simulink model "HVAC_ROS2_SafeSetpoint_v1"  (R2022b)
settings: Solver=FixedStepDiscrete  StartTime=0  StopTime=75  FixedStep=0.1  RelTol=1e-3
libraries: ros2lib x17
settings Model: Creator=Utilisateur  LastModifiedBy=Utilisateur
settings DataIOCC: ReturnWorkspaceOutputs=off
settings OptimizationCC: UseDivisionForNetSlopeComputation=on

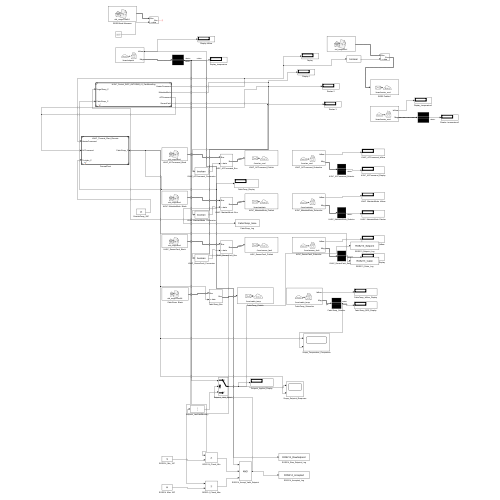
[thumbnail: Simulink's stored preview of the top-level diagram]
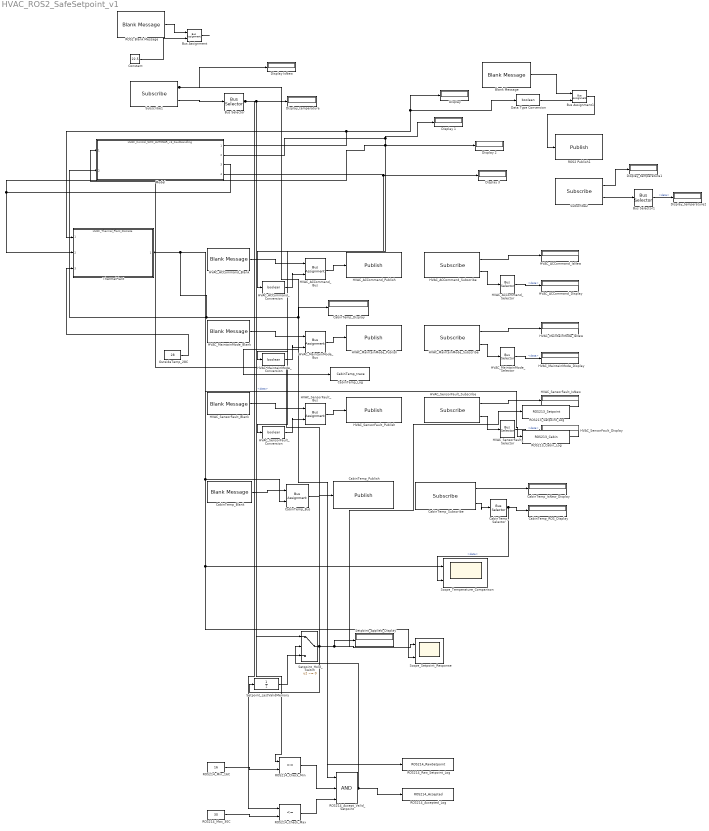
== system HVAC_ROS2_SafeSetpoint_v1 ==
  Blank Message : ros2lib/Blank Message  messageClass=Message  entityType=std_msgs/Bool  messageType=std_msgs/Bool  SampleTime=0.1
      settings: LibrarySourceBlock=roslib/ROS 2/Blank Message
  Bus Assignment : BusAssignment  AssignedSignals=data
  Bus Assignment1 : BusAssignment  AssignedSignals=data
  Bus Selector : BusSelector  OutputSignals=data
  Bus Selector1 : BusSelector  OutputSignals=data
  CabinTemp_Blank : ros2lib/Blank Message  messageClass=Message  entityType=std_msgs/Float64  messageType=std_msgs/Float64  SampleTime=0.1
      settings: LibrarySourceBlock=roslib/ROS 2/Blank Message
  CabinTemp_Bus : BusAssignment  AssignedSignals=data
  CabinTemp_Display : Display
  CabinTemp_IsNew_Display : Display
  CabinTemp_Log : ToWorkspace  VariableName=CabinTemp_trace  SaveFormat=Timeseries  SampleTime=-1
  CabinTemp_Publish : ros2lib/Publish  topicSource=Select from ROS network  topic=/hvac/cabin_temp  messageType=std_msgs/Float64  QOSHistory=Keep last  QOSDepth=1  QOSReliability=Reliable  QOSDurability=Volatile
      settings: LibrarySourceBlock=roslib/ROS 2/Publish
  CabinTemp_ROS_Display : Display
  CabinTemp_Selector : BusSelector  OutputSignals=data
  CabinTemp_Subscribe : ros2lib/Subscribe  topicSource=Specify your own  topic=/hvac/cabin_temp  messageType=std_msgs/Float64  sampleTime=0.1  QOSHistory=Keep last  QOSDepth=1  QOSReliability=Reliable  QOSDurability=Volatile
      settings: LibrarySourceBlock=roslib/ROS 2/Subscribe
  Constant : Constant  Value=22.5
  Data Type Conversion : DataTypeConversion  OutDataTypeStr=boolean  SaturateOnIntegerOverflow=off  RndMeth=Floor
  Display {,1..3} (4 alike) : Display
  Display IsNew : Display
  Display_temperature : Display
  Display_temperature1 : Display
  Display_temperature2 : Display
  HVAC_ACCommand_Blank : ros2lib/Blank Message  messageClass=Message  entityType=std_msgs/Bool  messageType=std_msgs/Bool  SampleTime=0.1
      settings: LibrarySourceBlock=roslib/ROS 2/Blank Message
  HVAC_ACCommand_Bus : BusAssignment  AssignedSignals=data
  HVAC_ACCommand_Conversion : DataTypeConversion  OutDataTypeStr=boolean  SaturateOnIntegerOverflow=off  RndMeth=Floor
  HVAC_ACCommand_Display : Display
  HVAC_ACCommand_IsNew : Display
  HVAC_ACCommand_Publish : ros2lib/Publish  topicSource=Select from ROS network  topic=/hvac/ac_cmd  messageType=std_msgs/Bool  QOSHistory=Keep last  QOSDepth=1  QOSReliability=Reliable  QOSDurability=Volatile
      settings: LibrarySourceBlock=roslib/ROS 2/Publish
  HVAC_ACCommand_Selector : BusSelector  OutputSignals=data
  HVAC_ACCommand_Subscribe : ros2lib/Subscribe  topicSource=Specify your own  topic=/hvac/ac_cmd  messageType=std_msgs/Bool  sampleTime=0.1  QOSHistory=Keep last  QOSDepth=1  QOSReliability=Reliable  QOSDurability=Volatile
      settings: LibrarySourceBlock=roslib/ROS 2/Subscribe
  HVAC_MaintainMode_Blank : ros2lib/Blank Message  messageClass=Message  entityType=std_msgs/Bool  messageType=std_msgs/Bool  SampleTime=0.1
      settings: LibrarySourceBlock=roslib/ROS 2/Blank Message
  HVAC_MaintainMode_Bus : BusAssignment  AssignedSignals=data
  HVAC_MaintainMode_Conversion : DataTypeConversion  OutDataTypeStr=boolean  SaturateOnIntegerOverflow=off  RndMeth=Floor
  HVAC_MaintainMode_Display : Display
  HVAC_MaintainMode_IsNew : Display
  HVAC_MaintainMode_Publish : ros2lib/Publish  topicSource=Select from ROS network  topic=/hvac/maintain  messageType=std_msgs/Bool  QOSHistory=Keep last  QOSDepth=1  QOSReliability=Reliable  QOSDurability=Volatile
      settings: LibrarySourceBlock=roslib/ROS 2/Publish
  HVAC_MaintainMode_Selector : BusSelector  OutputSignals=data
  HVAC_MaintainMode_Subscribe : ros2lib/Subscribe  topicSource=Specify your own  topic=/hvac/maintain  messageType=std_msgs/Bool  sampleTime=0.1  QOSHistory=Keep last  QOSDepth=1  QOSReliability=Reliable  QOSDurability=Volatile
      settings: LibrarySourceBlock=roslib/ROS 2/Subscribe
  HVAC_SensorFault_Blank : ros2lib/Blank Message  messageClass=Message  entityType=std_msgs/Bool  messageType=std_msgs/Bool  SampleTime=0.1
      settings: LibrarySourceBlock=roslib/ROS 2/Blank Message
  HVAC_SensorFault_Bus : BusAssignment  AssignedSignals=data
  HVAC_SensorFault_Conversion : DataTypeConversion  OutDataTypeStr=boolean  SaturateOnIntegerOverflow=off  RndMeth=Floor
  HVAC_SensorFault_Display : Display
  HVAC_SensorFault_IsNew : Display
  HVAC_SensorFault_Publish : ros2lib/Publish  topicSource=Select from ROS network  topic=/hvac/sensor_fault  messageType=std_msgs/Bool  QOSHistory=Keep last  QOSDepth=1  QOSReliability=Reliable  QOSDurability=Volatile
      settings: LibrarySourceBlock=roslib/ROS 2/Publish
  HVAC_SensorFault_Selector : BusSelector  OutputSignals=data
  HVAC_SensorFault_Subscribe : ros2lib/Subscribe  topicSource=Specify your own  topic=/hvac/sensor_fault  messageType=std_msgs/Bool  sampleTime=0.1  QOSHistory=Keep last  QOSDepth=1  QOSReliability=Reliable  QOSDurability=Volatile
      settings: LibrarySourceBlock=roslib/ROS 2/Subscribe
  Model : ModelReference  ModelNameDialog=HVAC_Control_SWC_AUTOSAR_v3_FaultHandling.slx  SimulationMode=Normal  ModelReferenceVersion=1.18
  OutsideTemp_28C : Constant  Value=28
  ROS2 Blank Message : ros2lib/Blank Message  messageClass=Message  entityType=std_msgs/Float64  messageType=std_msgs/Float64  SampleTime=0.1
      settings: LibrarySourceBlock=roslib/ROS 2/Blank Message
  ROS2 Publish1 : ros2lib/Publish  topicSource=Select from ROS network  topic=/hvac/heater_cmd  messageType=std_msgs/Bool  QOSHistory=Keep last  QOSDepth=1  QOSReliability=Reliable  QOSDurability=Volatile
      settings: LibrarySourceBlock=roslib/ROS 2/Publish
  ROS213_Cabin_Log : ToWorkspace  VariableName=ROS213_Cabin  SaveFormat=Timeseries  SampleTime=-1
  ROS213_Setpoint_Log : ToWorkspace  VariableName=ROS213_Setpoint  SaveFormat=Timeseries  SampleTime=-1
  ROS214_Accept_Valid_Setpoint : Logic  Inputs=3  AllPortsSameDT=off  OutDataTypeStr=boolean
  ROS214_Accepted_Log : ToWorkspace  VariableName=ROS214_Accepted  SaveFormat=Timeseries  SampleTime=-1
  ROS214_Check_Max : RelationalOperator  Operator=<=  OutDataTypeStr=boolean  RndMeth=Simplest  InputSameDT=off
  ROS214_Check_Min : RelationalOperator  OutDataTypeStr=boolean  RndMeth=Simplest  InputSameDT=off
  ROS214_Max_30C : Constant  Value=30
  ROS214_Min_16C : Constant  Value=16
  ROS214_Raw_Setpoint_Log : ToWorkspace  VariableName=ROS214_RawSetpoint  SaveFormat=Timeseries  SampleTime=-1
  Scope_Setpoint_Response : Scope  NumInputPorts=2
  Scope_Temperature_Comparison : Scope  NumInputPorts=2
  Setpoint_Applied_Display : Display
  Setpoint_Hold_Switch : Switch  Criteria=u2 ~= 0  SaturateOnIntegerOverflow=off  InputSameDT=off
  Setpoint_LastValidMemory : UnitDelay  InitialCondition=22.5  SampleTime=0.1  HasFrameUpgradeWarning=on
  Subscribe1 : ros2lib/Subscribe  topicSource=Specify your own  topic=/hvac/setpoint  messageType=std_msgs/Float64  sampleTime=0.1  QOSHistory=Keep last  QOSDepth=1  QOSReliability=Reliable  QOSDurability=Volatile
      settings: LibrarySourceBlock=roslib/ROS 2/Subscribe
  Subscribe2 : ros2lib/Subscribe  topicSource=Specify your own  topic=/hvac/heater_cmd  messageType=std_msgs/Bool  sampleTime=0.1  QOSHistory=Keep last  QOSDepth=1  QOSReliability=Reliable  QOSDurability=Volatile
      settings: LibrarySourceBlock=roslib/ROS 2/Subscribe
  ThermalPlant : ModelReference  ModelNameDialog=HVAC_Thermal_Plant_Discrete  SimulationMode=Normal  ModelReferenceVersion=1.2
  wires:
  Bus Assignment/1 -> ?
  Subscribe1/1 -> ROS214_Accept_Valid_Setpoint/1, Display IsNew/1
  ROS2 Blank Message/1 -> Bus Assignment/1
  Constant/1 -> Bus Assignment/2
  Subscribe1/2 -> Bus Selector/1
  Bus Selector/1 -> Display_temperature/1, Setpoint_Hold_Switch/1, ROS214_Check_Min/1, ROS214_Check_Max/1, ROS214_Raw_Setpoint_Log/1  "<data>"
  Model/1 -> "Display "/1, Data Type Conversion/1, ThermalPlant/1
  Model/2 -> Display 1/1, HVAC_MaintainMode_Conversion/1
  Model/3 -> Display 2/1, HVAC_ACCommand_Conversion/1, ThermalPlant/2
  Model/4 -> HVAC_SensorFault_Conversion/1, Display 3/1
  Data Type Conversion/1 -> Bus Assignment1/2
  Blank Message/1 -> Bus Assignment1/1
  Bus Assignment1/1 -> ROS2 Publish1/1
  Subscribe2/1 -> Display_temperature1/1
  Subscribe2/2 -> Bus Selector1/1
  Bus Selector1/1 -> Display_temperature2/1  "<data>"
  HVAC_ACCommand_Blank/1 -> HVAC_ACCommand_Bus/1
  HVAC_ACCommand_Conversion/1 -> HVAC_ACCommand_Bus/2
  HVAC_ACCommand_Bus/1 -> HVAC_ACCommand_Publish/1
  HVAC_ACCommand_Subscribe/1 -> HVAC_ACCommand_IsNew/1
  HVAC_ACCommand_Subscribe/2 -> HVAC_ACCommand_Selector/1
  HVAC_ACCommand_Selector/1 -> HVAC_ACCommand_Display/1  "<data>"
  HVAC_MaintainMode_Blank/1 -> HVAC_MaintainMode_Bus/1
  HVAC_MaintainMode_Conversion/1 -> HVAC_MaintainMode_Bus/2
  HVAC_MaintainMode_Bus/1 -> HVAC_MaintainMode_Publish/1
  HVAC_MaintainMode_Subscribe/1 -> HVAC_MaintainMode_IsNew/1
  HVAC_MaintainMode_Subscribe/2 -> HVAC_MaintainMode_Selector/1
  HVAC_MaintainMode_Selector/1 -> HVAC_MaintainMode_Display/1  "<data>"
  HVAC_SensorFault_Blank/1 -> HVAC_SensorFault_Bus/1
  HVAC_SensorFault_Conversion/1 -> HVAC_SensorFault_Bus/2
  HVAC_SensorFault_Bus/1 -> HVAC_SensorFault_Publish/1
  HVAC_SensorFault_Subscribe/1 -> HVAC_SensorFault_IsNew/1
  HVAC_SensorFault_Subscribe/2 -> HVAC_SensorFault_Selector/1
  HVAC_SensorFault_Selector/1 -> HVAC_SensorFault_Display/1  "<data>"
  OutsideTemp_28C/1 -> ThermalPlant/3
  ThermalPlant/1 -> Scope_Temperature_Comparison/1, Scope_Setpoint_Response/2, CabinTemp_Bus/2, CabinTemp_Log/1, CabinTemp_Display/1, Model/2, ROS213_Cabin_Log/1
  CabinTemp_Blank/1 -> CabinTemp_Bus/1
  CabinTemp_Bus/1 -> CabinTemp_Publish/1
  CabinTemp_Subscribe/2 -> CabinTemp_Selector/1
  CabinTemp_Selector/1 -> CabinTemp_ROS_Display/1, Scope_Temperature_Comparison/2  "<data>"
  CabinTemp_Subscribe/1 -> CabinTemp_IsNew_Display/1
  Setpoint_LastValidMemory/1 -> Setpoint_Hold_Switch/3
  Setpoint_Hold_Switch/1 -> Setpoint_Applied_Display/1, Scope_Setpoint_Response/1, Setpoint_LastValidMemory/1, Model/1, ROS213_Setpoint_Log/1
  ROS214_Min_16C/1 -> ROS214_Check_Min/2
  ROS214_Max_30C/1 -> ROS214_Check_Max/2
  ROS214_Check_Min/1 -> ROS214_Accept_Valid_Setpoint/2
  ROS214_Check_Max/1 -> ROS214_Accept_Valid_Setpoint/3
  ROS214_Accept_Valid_Setpoint/1 -> Setpoint_Hold_Switch/2, ROS214_Accepted_Log/1
